simulink model "ControlA"  (R2024b)
settings: Solver=VariableStepAuto  StartTime=0.0  StopTime=120  RelTol=1e-3
InitFcn:
  | run("circeuler")
StopFcn:
  | run("VidControlA.m")
settings Model: Creator=mery  LastModifiedBy=genni

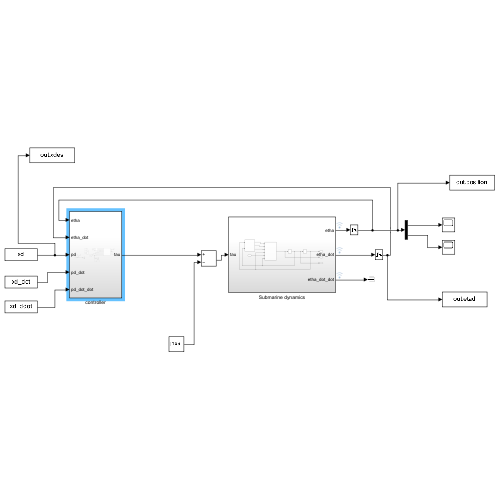
[thumbnail: Simulink's stored preview of the top-level diagram]
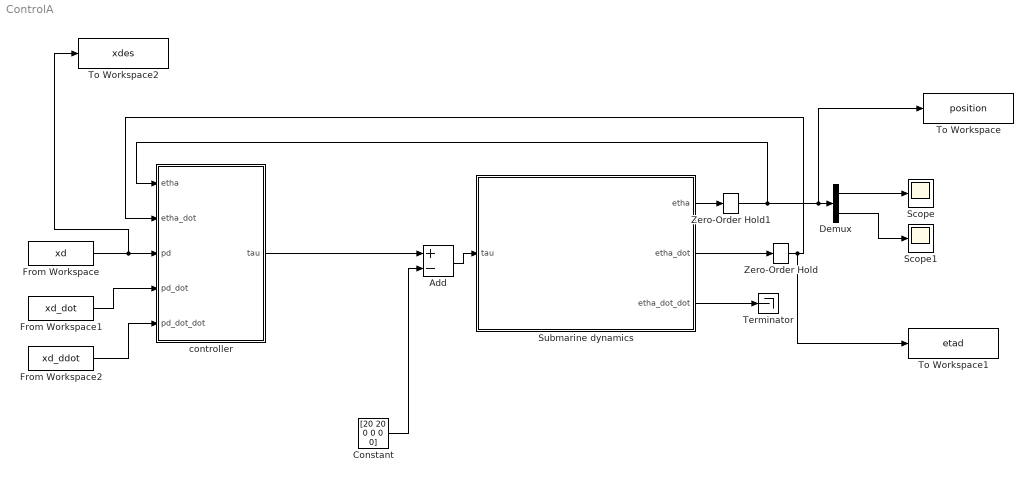
== system ControlA ==
  Add : Sum  Inputs=+-
  Constant : Constant  Value=[20 20 0 0 0 0]
  Demux : Demux  Outputs=2
  From Workspace : FromWorkspace  VariableName=xd  SampleTime=0.001
  From Workspace1 : FromWorkspace  VariableName=xd_dot  SampleTime=0.001
  From Workspace2 : FromWorkspace  VariableName=xd_ddot  SampleTime=0.001
  Scope : Scope
  Scope1 : Scope
  Submarine dynamics : Subsystem
  Terminator : Terminator
  To Workspace : ToWorkspace  VariableName=position  SaveFormat=Timeseries  SampleTime=-1
  To Workspace1 : ToWorkspace  VariableName=etad  SaveFormat=Timeseries  SampleTime=-1
  To Workspace2 : ToWorkspace  VariableName=xdes  SaveFormat=Timeseries  SampleTime=-1
  Zero-Order Hold : ZeroOrderHold  SampleTime=0.001
  Zero-Order Hold1 : ZeroOrderHold  SampleTime=0.001
  controller : Subsystem
  wires:
  Submarine dynamics/1(etha) -> Zero-Order Hold1/1
  Submarine dynamics/2(etha_dot) -> Zero-Order Hold/1
  Submarine dynamics/3(etha_dot_dot) -> Terminator/1
  From Workspace/1 -> To Workspace2/1, controller/3(pd)
  From Workspace2/1 -> controller/5(pd_dot_dot)
  From Workspace1/1 -> controller/4(pd_dot)
  Zero-Order Hold/1 -> To Workspace1/1, controller/2(etha_dot)
  Zero-Order Hold1/1 -> To Workspace/1, Demux/1, controller/1(etha)
  Demux/1 -> Scope/1
  Demux/2 -> Scope1/1
  controller/1(tau) -> Add/1
  Add/1 -> Submarine dynamics/1(tau)
  Constant/1 -> Add/2

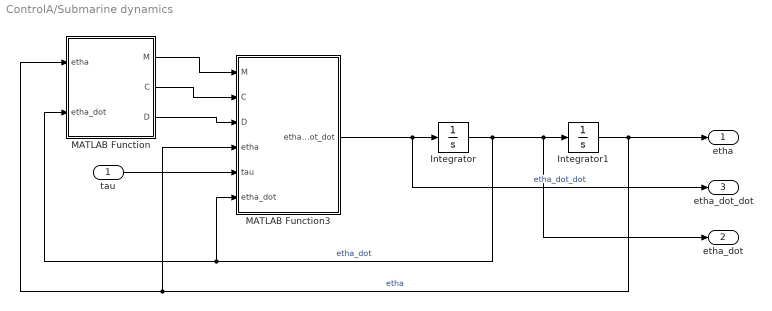
== system ControlA/Submarine dynamics ==
  tau : Inport
  Integrator : Integrator  InitialCondition=[0; 0; 0; 0; 0; 0]
  Integrator1 : Integrator  InitialCondition=[1; 0; 0; 0; 0; 0]
  MATLAB Function : MATLAB Function  TreatAsAtomicUnit=on
  MATLAB Function3 : MATLAB Function  TreatAsAtomicUnit=on
  etha : Outport
  etha_dot : Outport  Port=2
  etha_dot_dot : Outport  Port=3
  wires:
  Integrator/1 -> MATLAB Function/2(etha_dot), MATLAB Function3/6(etha_dot), etha_dot/1, Integrator1/1  "etha_dot"
  MATLAB Function/1(M) -> MATLAB Function3/1(M)
  MATLAB Function/2(C) -> MATLAB Function3/2(C)
  MATLAB Function/3(D) -> MATLAB Function3/3(D)
  MATLAB Function3/1(etha_dot_dot) -> etha_dot_dot/1, Integrator/1  "etha_dot_dot"
  Integrator1/1 -> etha/1, MATLAB Function/1(etha), MATLAB Function3/4(etha)  "etha"
  tau/1 -> MATLAB Function3/5(tau)

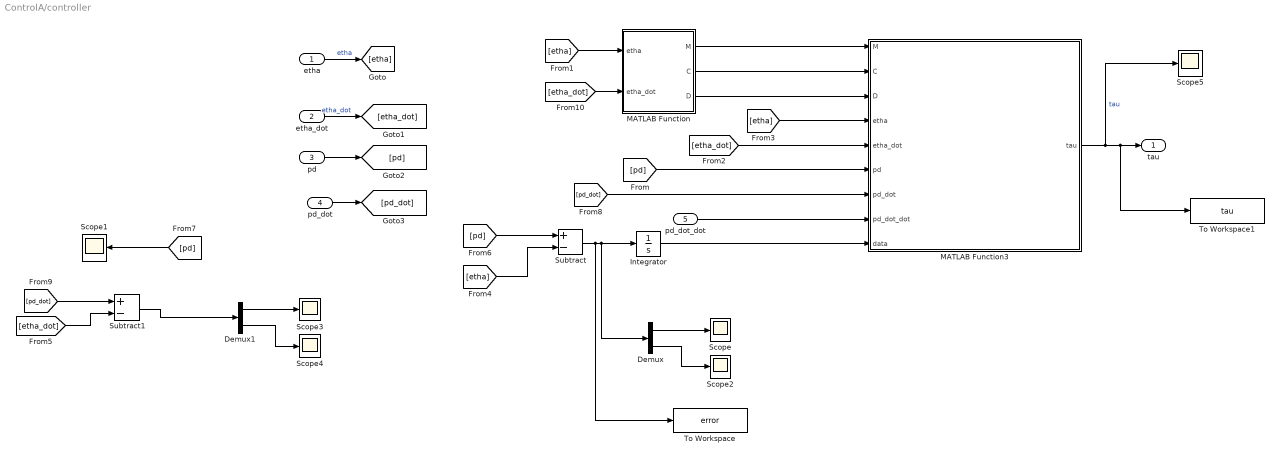
== system ControlA/controller ==
  etha : Inport
  etha_dot : Inport  Port=2
  pd : Inport  Port=3
  pd_dot : Inport  Port=4
  pd_dot_dot : Inport  Port=5
  Demux : Demux  Outputs=2
  Demux1 : Demux  Outputs=2
  Integrator : Integrator  InitialCondition=[1;0;0;0;0;0]
  MATLAB Function : MATLAB Function  TreatAsAtomicUnit=on
  MATLAB Function3 : MATLAB Function  TreatAsAtomicUnit=on
  Scope{,1..5} (6 alike) : Scope
  Subtract : Sum  Inputs=+-
  Subtract1 : Sum  Inputs=+-
  To Workspace : ToWorkspace  VariableName=error  SaveFormat=Timeseries  SampleTime=-1
  To Workspace1 : ToWorkspace  VariableName=tau  SaveFormat=Timeseries  SampleTime=-1
  tau : Outport
  wires:
  MATLAB Function/2(C) -> MATLAB Function3/2(C)
  MATLAB Function/1(M) -> MATLAB Function3/1(M)
  MATLAB Function/3(D) -> MATLAB Function3/3(D)
  MATLAB Function3/1(tau) -> Scope5/1, To Workspace1/1, tau/1  "tau"
  pd_dot_dot/1 -> MATLAB Function3/8(pd_dot_dot)
  Integrator/1 -> MATLAB Function3/9(data)
  Demux/2 -> Scope2/1
  Subtract/1 -> To Workspace/1, Demux/1, Integrator/1
  Demux/1 -> Scope/1
  Demux1/2 -> Scope4/1
  Demux1/1 -> Scope3/1
  Subtract1/1 -> Demux1/1
  etha/1 -> [etha]  "etha"
  [etha] -> MATLAB Function/1(etha)
  [etha] -> MATLAB Function3/4(etha)
  [etha] -> Subtract/2
  etha_dot/1 -> [etha_dot]  "etha_dot"
  [etha_dot] -> MATLAB Function3/5(etha_dot)
  [etha_dot] -> Subtract1/2
  pd/1 -> [pd]
  [pd] -> MATLAB Function3/6(pd)
  [pd] -> Subtract/1
  [pd] -> Scope1/1
  pd_dot/1 -> [pd_dot]
  [pd_dot] -> MATLAB Function3/7(pd_dot)
  [pd_dot] -> Subtract1/1
  [etha_dot] -> MATLAB Function/2(etha_dot)

== matlab function ControlA/controller/MATLAB Function ==
  data: etha input; M output; C output; D output; etha_dot input
function [M,C,D] = fcn(etha,etha_dot)

etha2=etha(4:6);

theta=etha2(2);
phi=etha2(1);
psi=etha2(3);

R_BI=[cos(psi)*cos(theta) sin(psi)*cos(theta) -sin(theta)
    -sin(psi)*cos(phi)+cos(psi)*sin(theta)*sin(phi) cos(psi)*cos(phi)+sin(psi)*sin(theta)*sin(phi) sin(phi)*cos(theta)
    sin(psi)*sin(phi)+cos(psi)*sin(theta)*cos(phi) -cos(psi)*sin(phi)+sin(psi)*sin(theta)*cos(phi) cos(phi)*cos(theta)];

J_k0=[1 0 -sin(theta)
    0 cos(phi) cos(theta)*sin(phi)
    0 -sin(phi) -cos(theta)*sin(phi)];

J_e=[R_BI zeros(3,3)
    zeros(3,3) J_k0];

ni=J_e*etha_dot;

u1=ni(1:3);
u2=ni(4:6);
a=0.6;
b=0.3;
c=0.3;
e_c=0.75;
mass=225;
g=9.81;
r_g=[0 0 0]';
r_b=[0 0 0.05]';
W=mass*g;
B=2219;
I_0=[8 0 0
    0 20 0
    0 0 20];
M_rb=[mass*eye(3) -mass*skew(r_g)
    mass*skew(r_g) I_0];

X_u_dot=-67;
Y_v_dot=-140;
Z_w_dot=-140;
K_p_dot=0;
M_q_dot=-2.5;
N_r_dot=-2.5;

M_a=diag([-X_u_dot -Y_v_dot -Z_w_dot -K_p_dot -M_q_dot -N_r_dot]);

M=M_rb+M_a;

C_rb=[zeros(3) -mass*skew(u1)-mass*skew(skew(u2)*r_g);
    -mass*skew(u1)-mass*skew(skew(u2)*r_g) mass*skew(skew(u2)*r_g)-skew(I_0*u2)];

u=u1(1);
v=u1(2);
w=u1(3);

p=u2(1);
q=u2(2);
r=u2(3);

C_a=[0 0 0 0 -Z_w_dot*w Y_v_dot*v
    0 0 0 Z_w_dot*w 0 -X_u_dot*u
    0 0 0 -Y_v_dot*v X_u_dot*u 0
    0 -Z_w_dot*w Y_v_dot*v 0 -N_r_dot*r M_q_dot*q
    Z_w_dot*w 0 -X_u_dot*u N_r_dot*r 0 -K_p_dot*p
    -Y_v_dot*v X_u_dot*u 0 -M_q_dot*q K_p_dot*p 0];

C=C_rb+C_a;

X_u_u=50;
Y_v_v=-100;
Z_w_w=-100;
K_p_p=-10;
M_q_q=-80;
N_r_r=-80;
K_p=-5;
M_q=-20;
N_r=-20;

D=diag([X_u_u*abs(u) -Y_v_v*abs(v) -Z_w_w*abs(w) -K_p-K_p_p*abs(p) -M_q-M_q_q*abs(q) -N_r-N_r_r*abs(r)]);

== matlab function ControlA/Submarine dynamics/MATLAB Function ==
  data: etha input; M output; C output; D output; etha_dot input
function [M,C,D] = fcn(etha,etha_dot)

etha2=etha(4:6);

theta=etha2(2);
phi=etha2(1);
psi=etha2(3);


R_BI=[cos(psi)*cos(theta) sin(psi)*cos(theta) -sin(theta)
    -sin(psi)*cos(phi)+cos(psi)*sin(theta)*sin(phi) cos(psi)*cos(phi)+sin(psi)*sin(theta)*sin(phi) sin(phi)*cos(theta)
    sin(psi)*sin(phi)+cos(psi)*sin(theta)*cos(phi) -cos(psi)*sin(phi)+sin(psi)*sin(theta)*cos(phi) cos(phi)*cos(theta)];

J_k0=[1 0 -sin(theta)
    0 cos(phi) cos(theta)*sin(phi)
    0 -sin(phi) -cos(theta)*sin(phi)];

J_e=[R_BI zeros(3,3)
    zeros(3,3) J_k0];

ni=J_e*etha_dot;

u1=ni(1:3);
u2=ni(4:6);
a=0.6;
b=0.3;
c=0.3;
e_c=0.75;
mass=225;
g=9.81;
r_g=[0 0 0]';
r_b=[0 0 0.05]';
W=mass*g;
B=2219;
I_0=[8 0 0
    0 20 0
    0 0 20];
M_rb=[mass*eye(3) -mass*skew(r_g)
    mass*skew(r_g) I_0];

X_u_dot=-67;
Y_v_dot=-140;
Z_w_dot=-140;
K_p_dot=0;
M_q_dot=-2.5;
N_r_dot=-2.5;

M_a=diag([-X_u_dot -Y_v_dot -Z_w_dot -K_p_dot -M_q_dot -N_r_dot]);

M=M_rb+M_a;

C_rb=[zeros(3) -mass*skew(u1)-mass*skew(skew(u2)*r_g);
    -mass*skew(u1)-mass*skew(skew(u2)*r_g) mass*skew(skew(u2)*r_g)-skew(I_0*u2)];

u=u1(1);
v=u1(2);
w=u1(3);

p=u2(1);
q=u2(2);
r=u2(3);

C_a=[0 0 0 0 -Z_w_dot*w Y_v_dot*v
    0 0 0 Z_w_dot*w 0 -X_u_dot*u
    0 0 0 -Y_v_dot*v X_u_dot*u 0
    0 -Z_w_dot*w Y_v_dot*v 0 -N_r_dot*r M_q_dot*q
    Z_w_dot*w 0 -X_u_dot*u N_r_dot*r 0 -K_p_dot*p
    -Y_v_dot*v X_u_dot*u 0 -M_q_dot*q K_p_dot*p 0];

C=C_rb+C_a;

X_u_u=-50;
Y_v_v=-100;
Z_w_w=-100;
K_p_p=-10;
M_q_q=-80;
N_r_r=-80;
K_p=-5;
M_q=-20;
N_r=-20;

D=diag([-X_u_u*abs(u) -Y_v_v*abs(v) -Z_w_w*abs(w) -K_p-K_p_p*abs(p) -M_q-M_q_q*abs(q) -N_r-N_r_r*abs(r)]);

== matlab function ControlA/controller/MATLAB Function3 ==
  data: M input; tau output; C input; D input; etha input; etha_dot input; pd input; pd_dot input; pd_dot_dot input; data input
function tau = fcn(M, C, D,etha,etha_dot,pd,pd_dot, pd_dot_dot, data)

etha2=etha(4:6);

theta=etha2(2);
phi=etha2(1);
psi=etha2(3);

etha2_dot=etha_dot(4:6);

theta_dot=etha2_dot(2);
phi_dot=etha2_dot(1);
psi_dot=etha2_dot(3);

R_BI=[cos(psi)*cos(theta) sin(psi)*cos(theta) -sin(theta)
    -sin(psi)*cos(phi)+cos(psi)*sin(theta)*sin(phi) cos(psi)*cos(phi)+sin(psi)*sin(theta)*sin(phi) sin(phi)*cos(theta)
    sin(psi)*sin(phi)+cos(psi)*sin(theta)*cos(phi) -cos(psi)*sin(phi)+sin(psi)*sin(theta)*cos(phi) cos(phi)*cos(theta)];

J_k0=[1 0 -sin(theta)
    0 cos(phi) cos(theta)*sin(phi)
    0 -sin(phi) cos(theta)*cos(phi)];

J_e=[R_BI zeros(3,3)
    zeros(3,3) J_k0];

J_e_inv=inv(J_e);

M_star= J_e_inv'*M*J_e_inv;

r11_dot = -sin(psi)*cos(theta)*psi_dot - cos(psi)*sin(theta)*theta_dot;
r12_dot =  cos(psi)*cos(theta)*psi_dot - sin(psi)*sin(theta)*theta_dot;
r13_dot = -cos(theta)*theta_dot;

r21_dot = -cos(psi)*cos(phi)*psi_dot ...
              - sin(psi)*sin(theta)*cos(phi)*psi_dot ...
              + sin(psi)*cos(theta)*sin(phi)*theta_dot ...
              + cos(psi)*sin(theta)*cos(phi)*phi_dot ...
              + cos(psi)*cos(theta)*sin(phi)*theta_dot;

    r22_dot = -sin(psi)*cos(phi)*psi_dot ...
              + cos(psi)*sin(theta)*cos(phi)*psi_dot ...
              + cos(psi)*cos(theta)*sin(phi)*theta_dot ...
              + sin(psi)*sin(theta)*cos(phi)*phi_dot ...
              + sin(psi)*cos(theta)*sin(phi)*theta_dot;

    r23_dot = -sin(phi)*cos(theta)*phi_dot - sin(phi)*sin(theta)*theta_dot;

    r31_dot =  cos(psi)*sin(phi)*psi_dot ...
              + sin(psi)*cos(phi)*phi_dot ...
              + cos(psi)*cos(theta)*cos(phi)*theta_dot ...
              - cos(psi)*sin(theta)*sin(phi)*phi_dot;

    r32_dot =  sin(psi)*sin(phi)*psi_dot ...
              - cos(psi)*cos(phi)*phi_dot ...
              + sin(psi)*cos(theta)*cos(phi)*theta_dot ...
              - sin(psi)*sin(theta)*sin(phi)*phi_dot;

    r33_dot = -sin(phi)*cos(theta)*phi_dot - cos(phi)*sin(theta)*theta_dot;

    R_dot = [r11_dot, r12_dot, r13_dot;
             r21_dot, r22_dot, r23_dot;
             r31_dot, r32_dot, r33_dot];

     % Derivata della matrice J_k0
    Jk0_dot = [0, 0, -cos(theta)*theta_dot;
               0, -sin(phi)*phi_dot, -sin(theta)*sin(phi)*theta_dot + cos(theta)*cos(phi)*phi_dot;
               0, -cos(phi)*phi_dot,  sin(theta)*sin(phi)*theta_dot - cos(theta)*cos(phi)*phi_dot];

    % Derivata della Jacobiana estesa Je
    Je_dot = [R_dot, zeros(3,3);
              zeros(3,3), Jk0_dot];

C_star=J_e_inv'*(C-M*J_e_inv*Je_dot)*J_e_inv;

D_star= J_e_inv'*D*J_e_inv;

g=9.81;
mass=225;
B=2219;
W=mass*g;

f_g=R_BI*[0;0;W];

f_b=-R_BI*[0;0;B];

r_g=[0 0 0]';
r_b=[0 0 0.05]';

g_RB=-[f_g+f_b
    cross(r_b,f_g)+cross(r_g,f_b)];

g_RB_star= J_e_inv'*g_RB;


Kp=diag([120*[3.5 2 2],[70 60 60]]);

Kd=diag([150*[1.5 1 1.5],90*[1 1 1]]);

KI=diag([40*[1 1 1],100*[1 1 1]]);
%KI=0;

pr_dot_dot=Kd*pd_dot_dot+Kp*(pd_dot-etha_dot)+KI*(pd-etha);

pr_dot=Kd*pd_dot+Kp*(pd-etha)+KI*data;

Lamda=170;

s=pr_dot-Kd*etha_dot;

%tau=M_star*pr_dot_dot+C_star*pr_dot+D_star*pr_dot+g_RB_star+Lamda*s;
 tau=g_RB_star+Lamda*s;

== matlab function ControlA/Submarine dynamics/MATLAB Function3 ==
  data: M input; etha_dot_dot output; C input; D input; etha input; tau input; etha_dot input
function etha_dot_dot = fcn(M, C, D,etha,tau,etha_dot)

etha2=etha(4:6);

theta=etha2(2);
phi=etha2(1);
psi=etha2(3);

etha2_dot=etha_dot(4:6);

theta_dot=etha2_dot(2);
phi_dot=etha2_dot(1);
psi_dot=etha2_dot(3);

R_BI=[cos(psi)*cos(theta) sin(psi)*cos(theta) -sin(theta)
    -sin(psi)*cos(phi)+cos(psi)*sin(theta)*sin(phi) cos(psi)*cos(phi)+sin(psi)*sin(theta)*sin(phi) sin(phi)*cos(theta)
    sin(psi)*sin(phi)+cos(psi)*sin(theta)*cos(phi) -cos(psi)*sin(phi)+sin(psi)*sin(theta)*cos(phi) cos(phi)*cos(theta)];

J_k0=[1 0 -sin(theta)
    0 cos(phi) cos(theta)*sin(phi)
    0 -sin(phi) cos(theta)*cos(phi)];

J_e=[R_BI zeros(3,3)
    zeros(3,3) J_k0];

J_e_inv=inv(J_e);

M_star= J_e_inv'*M*J_e_inv;

r11_dot = -sin(psi)*cos(theta)*psi_dot - cos(psi)*sin(theta)*theta_dot;
r12_dot =  cos(psi)*cos(theta)*psi_dot - sin(psi)*sin(theta)*theta_dot;
r13_dot = -cos(theta)*theta_dot;

r21_dot = -cos(psi)*cos(phi)*psi_dot ...
              - sin(psi)*sin(theta)*cos(phi)*psi_dot ...
              + sin(psi)*cos(theta)*sin(phi)*theta_dot ...
              + cos(psi)*sin(theta)*cos(phi)*phi_dot ...
              + cos(psi)*cos(theta)*sin(phi)*theta_dot;

    r22_dot = -sin(psi)*cos(phi)*psi_dot ...
              + cos(psi)*sin(theta)*cos(phi)*psi_dot ...
              + cos(psi)*cos(theta)*sin(phi)*theta_dot ...
              + sin(psi)*sin(theta)*cos(phi)*phi_dot ...
              + sin(psi)*cos(theta)*sin(phi)*theta_dot;

    r23_dot = -sin(phi)*cos(theta)*phi_dot - sin(phi)*sin(theta)*theta_dot;

    r31_dot =  cos(psi)*sin(phi)*psi_dot ...
              + sin(psi)*cos(phi)*phi_dot ...
              + cos(psi)*cos(theta)*cos(phi)*theta_dot ...
              - cos(psi)*sin(theta)*sin(phi)*phi_dot;

    r32_dot =  sin(psi)*sin(phi)*psi_dot ...
              - cos(psi)*cos(phi)*phi_dot ...
              + sin(psi)*cos(theta)*cos(phi)*theta_dot ...
              - sin(psi)*sin(theta)*sin(phi)*phi_dot;

    r33_dot = -sin(phi)*cos(theta)*phi_dot - cos(phi)*sin(theta)*theta_dot;

    R_dot = [r11_dot, r12_dot, r13_dot;
             r21_dot, r22_dot, r23_dot;
             r31_dot, r32_dot, r33_dot];

     % Derivata della matrice J_k0
    Jk0_dot = [0, 0, -cos(theta)*theta_dot;
               0, -sin(phi)*phi_dot, -sin(theta)*sin(phi)*theta_dot + cos(theta)*cos(phi)*phi_dot;
               0, -cos(phi)*phi_dot,  sin(theta)*sin(phi)*theta_dot - cos(theta)*cos(phi)*phi_dot];

    % Derivata della Jacobiana estesa Je
    Je_dot = [R_dot, zeros(3,3);
              zeros(3,3), Jk0_dot];

C_star=J_e_inv'*(C-M*J_e_inv*Je_dot)*J_e_inv;

D_star= J_e_inv'*D*J_e_inv;

g=9.81;
mass=225;
B=2219;
W=mass*g;

f_g=R_BI*[0;0;W];

f_b=-R_BI*[0;0;B];

r_g=[0 0 0]';
r_b=[0 0 0.05]';

g_RB=-[f_g+f_b
    cross(r_b,f_g)+cross(r_g,f_b)];

g_RB_star= J_e_inv'*g_RB;

% tau_star= J_e_inv'*tau;
tau_star= tau;

inversa=inv(M_star);

etha_dot_dot=inversa*(tau_star-C_star*etha_dot-D_star*etha_dot-g_RB_star);
